simulink model "twiddle_general_4mult_test"  (Simulink 7.2)
settings: Solver=VariableStepDiscrete  StartTime=0.0  StopTime=1000  RelTol=1e-3
libraries: xbsIndex_r4 x27, casper_library_misc x5, simulink x1
settings Model: Creator=User  LastModifiedBy=root
settings OptimizationCC: InitFltsAndDblsToZero=on
settings DebuggingCC: SaveWithDisabledLinksMsg=none  SaveWithParameterizedLinksMsg=none

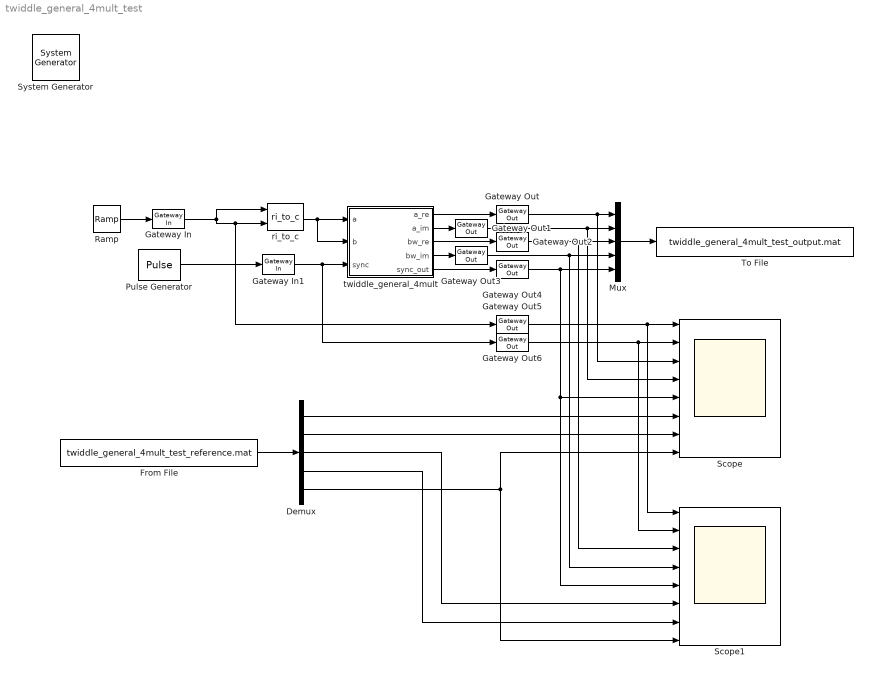
== system twiddle_general_4mult_test ==
  " System Generator" : xbsIndex_r4/ System Generator  Tag=genX  SystemSampleTime=-1  xilinxfamily=Virtex4  part=xc4vsx35  speed=-10  package=ff668  synthesis_tool=XST  clock_wrapper=Clock Enables  directory=./netlist  testbench=off  simulink_period=1  sysclk_period=100  dcm_input_clock_period=100  incr_netlist=off  trim_vbits=Everywhere in SubSystem  dbl_ovrd=According to Block Masks  core_generation=According to Block Masks  run_coregen=off  deprecated_control=off  eval_field=0  block_type=sysgen
      settings: block_version=10.1.1
  Demux : Demux  Outputs=5
  From File : FromFile  FileName=twiddle_general_4mult_test_reference.mat  SampleTime=1
  Gateway In : xbsIndex_r4/Gateway In  arith_type="Signed  (2's comp)"  n_bits=5  bin_pt=4  quantization=Truncate  overflow=Wrap  period=1  dbl_ovrd=off  timing_constraint=None  locs_specified=off  LOCs={}  hdl_port=on  block_type=gatewayin
      settings: infoedit="Gateway in block.  Converts inputs of type Simulink integer, double and fixed point to  Xilinx fixed point type.<P><P>Hardware notes:  In hardware these blocks become top level input ports."  block_version=10.1.1
  Gateway In1 : xbsIndex_r4/Gateway In  arith_type=Boolean  n_bits=16  bin_pt=14  quantization="Round  (unbiased: +/- Inf)"  overflow=Saturate  period=1  dbl_ovrd=off  timing_constraint=None  locs_specified=off  LOCs={}  hdl_port=on  block_type=gatewayin
      settings: infoedit="Gateway in block.  Converts inputs of type Simulink integer, double and fixed point to  Xilinx fixed point type.<P><P>Hardware notes:  In hardware these blocks become top level input ports."  block_version=10.1.1
  Gateway Out{,1..6} (7 alike) : xbsIndex_r4/Gateway Out  hdl_port=on  timing_constraint=None  locs_specified=off  LOCs={}  block_type=gatewayout
      settings: infoedit="Gateway out block.  Converts Xilinx fixed point inputs into ouputs of type Simulink integer, double, or fixed point.<P><P>Hardware notes:  In hardware these blocks become top level output ports or are discarded, depending on how they are configured."  block_version=10.1.1
  Mux : Mux  Inputs=5
  Pulse Generator : DiscretePulseGenerator  Period=256  PhaseDelay=7
  Ramp : simulink/Sources/Ramp  SystemSampleTime=-1  slope=1/2^5  start=0  X0=0
  Scope : Scope  NumInputPorts=8
      settings: TimeRange=1000  YMin=-1~0~-1~-1~0~-1~-1~-1  YMax=1~1~1~1~1~1~1~1
  Scope1 : Scope  NumInputPorts=8
      settings: YMin=-1~-1~-1~-1~-1~-1~-1~-1  YMax=1~1~1~1~1~1~1~1
  To File : ToFile  Filename=twiddle_general_4mult_test_output.mat  MatrixName=output
  ri_to_c : casper_library_misc/ri_to_c  SystemSampleTime=-1
  twiddle_general_4mult : Subsystem  AncestorBlock=casper_library_ffts_twiddle/twiddle_general_4mult  mask(twiddle_general_4mult){Coeffs=getfield( getfield( get_param( gcb,'UserData' ), 'parameters'),'Coeffs'), StepPeriod=1, coeffs_bram=on, coeff_bit_width=5, input_bit_width=5, add_latency=2, mult_latency=3, bram_latency=2, conv_latency=1, arch=Virtex2Pro, use_hdl=on, use_embedded=off, quantization=Round  (unbiased: +/- Inf), overflow=Wrap}
      mask prompts: Coeffs "Coefficients:"; StepPeriod "Coefficient Step Period (2^?)"; coeffs_bram "Store coefficients in BRAM"; coeff_bit_width "Coefficient Bit Width"; input_bit_width "Input Bit Width"; add_latency "Add Latency"; mult_latency "Mult Latency"; bram_latency "BRAM Latency"; conv_latency "Convert Latency"; arch "Architecture"; use_hdl "Use behavioural HDL for multipliers"; use_embedded "Use embedded multipliers"; quantization "Quantization Behavior"; overflow "Overflow Behavior"
      mask help:
      | Used in biplex pipelined FFT. Implements
      | (a+bi)(c+di) as (ac-bd)+i(ad+bc) with four
      | multipliers
      mask init:
      | twiddle_general_4mult_init(gcb, ...
      |     'Coeffs', Coeffs, ...
      |     'StepPeriod', StepPeriod, ...
      |     'coeffs_bram', coeffs_bram, ...
      |     'coeff_bit_width', coeff_bit_width, ...
      |     'input_bit_width', input_bit_width, ...
      |     'add_latency', add_latency, ...
      |     'mult_latency', mult_latency, ...
      |     'bram_latency', bram_latency, ...
      |     'conv_latency', conv_latency, ...
      |     'arch', arch, ...
      |     'use_hdl', use_hdl, ...
      |     'use_embedded', use_embedded, ...
      |     'quantization', quantization, ...
      |     'overflow', overflow)
      settings: AttributesFormatString=|
      | data=(5,4)
      | coeffs=(5,3)
      | Virtex2Pro
      | (Round  (unbiased: +/- Inf),Wrap)
      mask StyleString: edit,edit,checkbox,edit,edit,edit,edit,edit,edit,popup(Virtex2Pro|Virtex5),checkbox,checkbox,popup(Truncate|Round  (unbiased: +/- Inf)|Round  (unbiased: Even Values)),popup(Wrap|Saturate|Error)
      mask CallbackString:
      | ||||||||||use_hdl = get_param(gcb,'use_hdl');
      | visibs = get_param(gcb, 'MaskVisibilities');
      | if( strcmp(use_hdl,'on')),
      |     set_param(gcb, 'use_embedded','off');
      |     visibs{12} = 'off';
      | else,
      |     visibs{12} = 'on';
      | end
      | set_param(gcb, 'MaskVisibilities', visibs);|||
  wires:
  Ramp/1 -> Gateway In/1
  Pulse Generator/1 -> Gateway In1/1
  Gateway In1/1 -> Gateway Out6/1, twiddle_general_4mult/3(sync)
  twiddle_general_4mult/1(a_re) -> Gateway Out/1
  twiddle_general_4mult/2(a_im) -> Gateway Out1/1
  twiddle_general_4mult/3(bw_re) -> Gateway Out2/1
  twiddle_general_4mult/4(bw_im) -> Gateway Out3/1
  twiddle_general_4mult/5(sync_out) -> Gateway Out4/1
  Gateway Out/1 -> Mux/1, Scope/3
  Gateway Out1/1 -> Mux/2, Scope/4
  Gateway Out2/1 -> Mux/3, Scope1/3
  Gateway Out3/1 -> Mux/4, Scope1/4
  Gateway Out4/1 -> Mux/5, Scope/5, Scope1/5
  Mux/1 -> To File/1
  Gateway Out5/1 -> Scope/1, Scope1/1
  Gateway Out6/1 -> Scope/2, Scope1/2
  Gateway In/1 -> ri_to_c/1, ri_to_c/2, Gateway Out5/1
  ri_to_c/1 -> twiddle_general_4mult/1(a), twiddle_general_4mult/2(b)
  Demux/2 -> Scope/7
  Demux/5 -> Scope/8, Scope1/8
  Demux/1 -> Scope/6
  Demux/3 -> Scope1/6
  Demux/4 -> Scope1/7
  From File/1 -> Demux/1

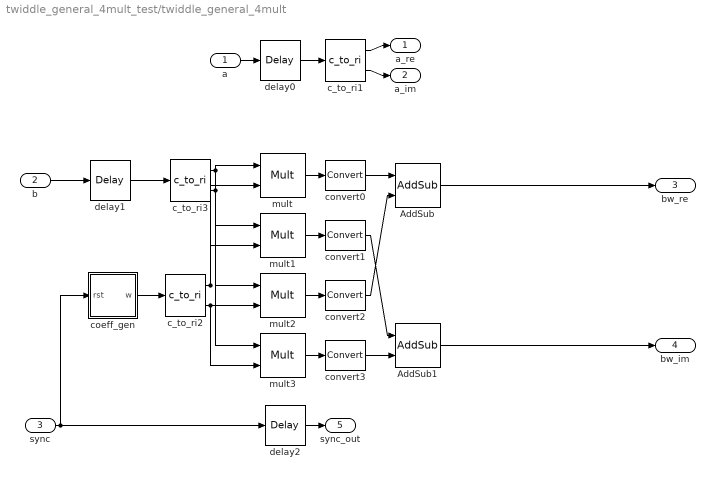
== system twiddle_general_4mult_test/twiddle_general_4mult ==
  a : Inport
  b : Inport  Port=2
  sync : Inport  Port=3
  AddSub : xbsIndex_r4/AddSub  mode=Subtraction  use_carryin=off  use_carryout=off  en=off  latency=add_latency  precision=Full  arith_type=Unsigned  n_bits=16  bin_pt=14  quantization=Truncate  overflow=Wrap  dbl_ovrd=off  use_behavioral_HDL=on  hw_selection=Fabric  pipelined=off  block_type=addsub
  AddSub1 : xbsIndex_r4/AddSub  mode=Addition  use_carryin=off  use_carryout=off  en=off  latency=add_latency  precision=Full  arith_type=Unsigned  n_bits=16  bin_pt=14  quantization=Truncate  overflow=Wrap  dbl_ovrd=off  use_behavioral_HDL=on  hw_selection=Fabric  pipelined=off  block_type=addsub
  c_to_ri1 : casper_library_misc/c_to_ri  SystemSampleTime=-1  n_bits=input_bit_width  bin_pt=input_bit_width-1
      settings: AttributesFormatString=5_4 r/i
  c_to_ri2 : casper_library_misc/c_to_ri  SystemSampleTime=-1  n_bits=coeff_bit_width  bin_pt=coeff_bit_width-2
      settings: AttributesFormatString=5_3 r/i
  c_to_ri3 : casper_library_misc/c_to_ri  SystemSampleTime=-1  n_bits=input_bit_width  bin_pt=input_bit_width-1
      settings: AttributesFormatString=5_4 r/i
  coeff_gen : Subsystem  AncestorBlock=casper_library_ffts_twiddle_coeff_gen/coeff_gen  mask(coeff_gen){Coeffs=getfield( getfield( get_param( gcb,'UserData' ), 'parameters'),'Coeffs'), coeff_bit_width=5, StepPeriod=1, bram_latency=2, coeffs_bram=on}
      mask prompts: Coeffs "Coefficients: (0 to 2^(FFTSize-1)-1)"; coeff_bit_width "Coefficient Bit Width:"; StepPeriod "Step Period: (2^?)"; bram_latency "Latency:"; coeffs_bram "Store coefficients in BRAM"
      mask help: Generates a sequence of complex coefficients
      mask init:
      | coeff_gen_init( gcb, ...
      |     'Coeffs', Coeffs, ...
      |     'coeff_bit_width', coeff_bit_width, ...
      |     'StepPeriod', StepPeriod, ...
      |     'bram_latency', bram_latency, ...
      |     'coeffs_bram', coeffs_bram);
      settings: AttributesFormatString=8 @ (5,3)
      mask CallbackString:
      | Coeffs = eval(get_param(gcb, 'Coeffs'));
      | if( length(Coeffs) == 1 ),
      |     set_param(gcb, 'MaskVisibilities',{'on','on','off','off','off'});
      | else
      |     set_param(gcb, 'MaskVisibilities',{'on','on','on','on','on'});
      | end||||
  convert{0..3} (4 alike) : xbsIndex_r4/Convert  arith_type="Signed  (2's comp)"  n_bits=input_bit_width+3  bin_pt=input_bit_width+1  quantization="Round  (unbiased: +/- Inf)"  overflow=Wrap  latency=conv_latency  dbl_ovrd=off  pipeline=on  block_type=convert
      settings: block_version=11.4
  delay0 : xbsIndex_r4/Delay  en=off  latency=mult_latency + add_latency + bram_latency + conv_latency  dbl_ovrd=off  reg_retiming=off  block_type=delay
      settings: block_version=11.4
  delay1 : xbsIndex_r4/Delay  en=off  latency=bram_latency  dbl_ovrd=off  reg_retiming=on  block_type=delay
      settings: block_version=11.4
  delay2 : xbsIndex_r4/Delay  en=off  latency=mult_latency + add_latency + bram_latency + conv_latency  dbl_ovrd=off  reg_retiming=off  block_type=delay
      settings: block_version=11.4
  mult{,1..3} (4 alike) : xbsIndex_r4/Mult  precision=Full  arith_type="Signed  (2's comp)"  n_bits=16  bin_pt=14  quantization=Truncate  overflow=Wrap  en=off  latency=mult_latency  dbl_ovrd=off  use_behavioral_HDL=on  opt=Speed  use_embedded=off  optimum_pipeline=off  pipeline=on  use_rpm=on  placement_style=Triangular  block_type=mult
      settings: block_version=11.4
  a_re : Outport
  a_im : Outport  Port=2
  bw_re : Outport  Port=3
  bw_im : Outport  Port=4
  sync_out : Outport  Port=5
  wires:
  a/1 -> delay0/1
  delay0/1 -> c_to_ri1/1
  c_to_ri1/1 -> a_re/1
  c_to_ri1/2 -> a_im/1
  sync/1 -> delay2/1, coeff_gen/1(rst)
  delay2/1 -> sync_out/1
  coeff_gen/1(w) -> c_to_ri2/1
  b/1 -> delay1/1
  delay1/1 -> c_to_ri3/1
  c_to_ri3/1 -> mult/1, mult3/1
  c_to_ri2/1 -> mult/2, mult1/2
  c_to_ri3/2 -> mult1/1, mult2/1
  c_to_ri2/2 -> mult2/2, mult3/2
  mult/1 -> convert0/1
  mult1/1 -> convert1/1
  mult2/1 -> convert2/1
  mult3/1 -> convert3/1
  convert0/1 -> AddSub/1
  convert2/1 -> AddSub/2
  convert1/1 -> AddSub1/1
  convert3/1 -> AddSub1/2
  AddSub/1 -> bw_re/1
  AddSub1/1 -> bw_im/1

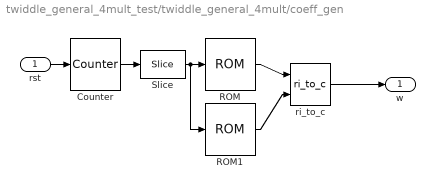
== system twiddle_general_4mult_test/twiddle_general_4mult/coeff_gen ==
  rst : Inport
  Counter : xbsIndex_r4/Counter  cnt_type=Free Running  cnt_to=Inf  operation=Up  start_count=0  cnt_by_val=1  arith_type=Unsigned  n_bits=4  bin_pt=0  load_pin=off  rst=on  en=off  explicit_period=on  period=1  dbl_ovrd=off  use_behavioral_HDL=off  implementation=Fabric  block_type=counter
      settings: block_version=11.4
  ROM : xbsIndex_r4/ROM  depth=8  initVector="[0                                      0                                  0.125                                  0.125                                   0.25                                   0.25                                   0.25                                  0.375]"  distributed_mem=Block RAM  rst=off  init_reg=0  en=off  latency=2  arith_type="Signed  (2's comp)"  n_bits=5  bin_pt=3  dbl_ovrd=off  optimize=Area  use_rpm=on  block_type=sprom
      settings: block_version=11.4
  ROM1 : xbsIndex_r4/ROM  depth=8  initVector="[-0                                 -0.125                                 -0.125                                  -0.25                                  -0.25                                  -0.25                                 -0.375                                 -0.375]"  distributed_mem=Block RAM  rst=off  init_reg=0  en=off  latency=2  arith_type="Signed  (2's comp)"  n_bits=5  bin_pt=3  dbl_ovrd=off  optimize=Area  use_rpm=on  block_type=sprom
      settings: block_version=11.4
  Slice : xbsIndex_r4/Slice  nbits=3  boolean_output=off  mode=Upper Bit Location + Width  bit1=0  base1=MSB of Input  bit0=0  base0=LSB of Input  dbl_ovrd=off  block_type=slice
  ri_to_c : casper_library_misc/ri_to_c  SystemSampleTime=-1
  w : Outport
  wires:
  ri_to_c/1 -> w/1
  rst/1 -> Counter/1
  Counter/1 -> Slice/1
  Slice/1 -> ROM/1, ROM1/1
  ROM/1 -> ri_to_c/1
  ROM1/1 -> ri_to_c/2
